simulink model "commhdlQPSKTxRx"  (R2025b)
settings: Solver=FixedStepDiscrete  StartTime=0.0  StopTime=stopTime  RelTol=1e-3
PostLoadFcn:
  | hScopeConfig = get_param([gcs '/Receiver/QPSK Rx/Frequency and Time Synchronizer/Symbol Synchronizer/No HDL/QPSK Receiver Eye Diagram'],'ScopeConfiguration');
  | 
  | hScopeConfig.OpenAtSimulationStart = false;
  | hScopeConfig.Visible = false;
  | SamplesPerSymbol = 4;
  | %UpsamplesRx = 1;
  | clear hScopeConfig
InitFcn:
  | commhdlQPSKTxRxModelInit;
  | % Rate bridge: ADRV9002/Jupiter radio runs at 15.36 MHz = 2x the 7.68 MHz
  | % (4 samples/symbol @ Rsym=1.92 MHz) the QPSK Rx requires. The deployed
  | % Receiver must downsample the ADC stream by 2. UpsamplesRx=1 fed the QPSK
  | % Rx 8 sps (2x-upsampled) and broke symbol sync / the loopback bit check.
  | UpsamplesRx = 1;   %% T8 RATE FIX: rail 15.36e6 == ADC bus rate,
  | %% no ingress decimation (was 2 when the rail sat on the 7.68e6 rung)
  | UpsamplesTx = 1;
  | clear simTimingOffset;
StopFcn:
  | if exist('simTimingOffset','var')
  |   disp('Simulation completed');
  |   %QPSKTxRxVerification;
  | end
undefined symbols (not defined in the file or in its folder): Add, Config, fsym, randsrc, RandStream, Rsym, Shift
libraries: hdlsllib x76, simulink x21, dspsigops x19, dsphdlfiltering2 x3, dsphdlsigops2 x2, dsphdlmathfun2 x2, commdigbbndpm3 x2, commchan3 x1, commrflib2 x1
(part 1 of 4)
CloseFcn:
  | clear Config CSLatency dataBits dataIn DBPP DescramblerLatency endLoc ...
  |         errSym errWaveform falsePacketsNo FCLatency idx initFramesNotToCompareInRx ...
  |         Nframes nReceivedBits PALatency PDLatency pktNo QPSKDemodLatency ...
  |         refQPSKSym refTxWaveform Rsym RxBits RxOut RxOutEnd RxOutSrt ...
  |         simAfterCS simBeforeSS simPeakFind simQPSKSym simSyncedPackets ...
  |         simTimingOffset simTxWaveform srtLoc SSLatency stopTime tout trueOffset ...
  |         TxBits validIn vPktNo
  | clear SamplesPerSymbol nErrBits nErrPkts nMissedPkts TxSymbolsMaxError TxWaveformMaxError
settings Model: DataTypeOverride=Off  Creator=The MathWorks, Inc.  LastModifiedBy=tcollins
settings SolverCC: AlgebraicLoopSolver=TrustRegion  MaxZcPerStep=1.0
settings DataIOCC: ReturnWorkspaceOutputs=off
settings OptimizationCC: BlockReduction=off  ConditionallyExecuteInputs=off  DefaultParameterBehavior=Inlined  ReuseModelBlockBuffer=off
settings DebuggingCC: AlgebraicLoopMsg=error  SingleTaskRateTransMsg=error  UnconnectedInputMsg=warning  UnconnectedOutputMsg=warning  UnconnectedLineMsg=warning  SubsystemReferenceDiagnosticForUnitTest=warning
settings HardwareCC: ProdBitPerPointer=32.0  ProdBitPerSizeT=32.0  ProdBitPerPtrDiffT=32.0  ProdLargestAtomicFloat=None  ProdIntDivRoundTo=Undefined  ProdEndianess=Unspecified  ProdWordSize=32.0  ProdHWDeviceType=ASIC/FPGA->ASIC/FPGA  TargetBitPerLong=64.0  TargetBitPerPointer=64.0  TargetBitPerSizeT=64.0  TargetBitPerPtrDiffT=64.0  TargetLongLongMode=on  TargetIntDivRoundTo=Zero  TargetEndianess=LittleEndian  TargetWordSize=64.0  TargetHWDeviceType=Custom Processor->MATLAB Host Computer  ProdEqTarget=off
settings ModelReferenceCC: EnableRefExpFcnMdlSchedulingChecks=on
settings RTWCC: GPUComputeCapability=3.5  DLArmComputeVersion=19.05

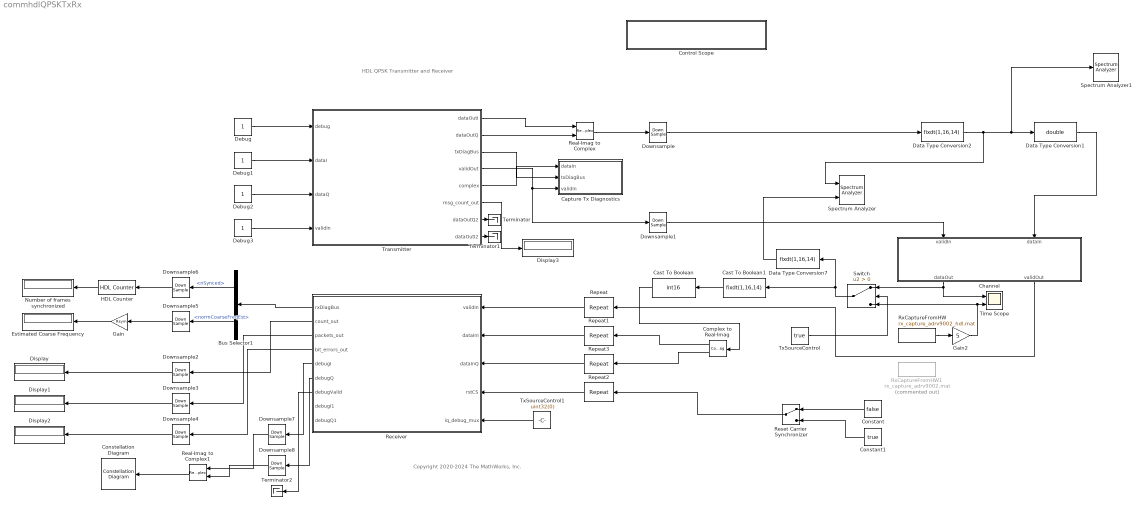
== system commhdlQPSKTxRx ==
  note: HDL QPSK Transmitter and Receiver
  note: Copyright 2020-2024 The MathWorks, Inc.
  Bus Selector1 : BusSelector  OutputSignals=nSynced,normCoarseFreqEst
  Capture Tx Diagnostics : Subsystem
  Cast To Boolean : DataTypeConversion  OutDataTypeStr=int16  ConvertRealWorld=Stored Integer (SI)  SaturateOnIntegerOverflow=off  RndMeth=Floor
  Cast To Boolean1 : DataTypeConversion  OutDataTypeStr=fixdt(1,16,14)  SaturateOnIntegerOverflow=off  RndMeth=Floor
  Channel : Subsystem  mask{EbN0dB=40, CFO=1e3, CPO=135, fractionalTimingOffset=0.55, timingFrequencyOffset=2}
      mask prompts: EbN0dB "Eb/N0 (in dB) :"; CFO "Carrier Frequency Offset (in Hz):"; CPO "Carrier Phase Offset (in Degrees) :"; fractionalTimingOffset "Fractional Timing Offset ( <1 ) :"; timingFrequencyOffset "Timing Frequency Offset (in PPM) :"
      mask init:
      | validateattributes(fractionalTimingOffset,{'double'},{'finite','scalar','nonnegative','>=',0,'<',1},'','fractionalTimingOffset');
      | validateattributes(timingFrequencyOffset,{'double'},{'finite','scalar','nonnegative'},'','timingFrequencyOffset');
      | validateattributes(EbN0dB,{'double'},{'scalar'},'','EbN0dB');
      | validateattributes(CFO,{'double'},{'finite','scalar',},'','CFO');
      | validateattributes(CPO,{'double'},{'finite','scalar'},'','CPO');
      | 
      | BitsPerSymbol = 2;      % QPSK
      | EbN0          = 10^(EbN0dB/10);
      | EsN0          = BitsPerSymbol*EbN0;
      | noiseVariance = 1/EsN0;  % QPSK symbol energy is normalized to 1 i.e. Es = 1
      | 
      | clear BitsPersymbol EbN0 EsN0
      settings: PortSchema="{\"entries\":[{\"content\":{\"sides\":[{\"content\":{\"connectorIds\":[]},\"type\":\"ConnectorPlacement.EquallySpacedRectSide\",\"uuid\":\"aa9ac445-3d73-401b-8e6c-a43fa6f53e3e\"},{\"content\":{\"connectorIds\":[],\"side\":\"RIGHT\"},\"type\":\"ConnectorPlacement.EquallySpacedRectSide\",\"uuid\":\"c8fbe2c1-ad18-4b81-8824-4fece19db9b5\"},{\"content\":{\"connectorIds\":[\"In1\",\"In2\"],\"side\":\"TOP\"},\"type\":\"ConnectorPlacement.EquallySpacedRectSide\",\"uuid\":\"2fdd8701-02b7-4a19-ab6e-54d2593732fa\"},{\"content\":{\"connectorIds\":[\"Out1\",\"Out2\"],\"side\":\"BOTTOM\"},\"type\":\"ConnectorPlacement.EquallySpacedRectSide\",\"uuid\":\"bd6ca111-71ba-47de-a918-1bcd41b09175\"}]},\"type\":\"ConnectorPlacement.EquallySpacedConnector\",\"uuid\":\"c410269f-5de3-4a8f-bc07-850237ff35fb\"}],\"packageUris\":[\"http://schema.mathworks.com/mf0/Connector/R2020b\"],\"version\":\"1.0\"}"
      mask DialogControl DescGroupVar Prompt: Channel
      mask Display: disp(['Double-Click' newline 'to set channel']);
  Complex to Real-Imag : ComplexToRealImag
  Constant : Constant  Value=false  SampleTime=1/(Rsym*Config.SamplesPerSymbol)
  Constant1 : Constant  Value=true  SampleTime=1/(Rsym*Config.SamplesPerSymbol)
  Constellation Diagram : ConstellationDiagram  WindowPosition=[594.000000,164.000000,600.000000,600.000000,]  Visible=on  ScopeFrameLocation=window  SymbolsToDisplaySource=Property  SymbolsToDisplay=1000  XLimits=[-1.375,8542.5]  YLimits=[-1.375,8542.5]  AxesLimits=[-1.375,8542.5]  MaximizeAxes=on  DefaultConfigurationName=comm.scopes.ConstellationDiagramBlockCfg
  Control Scope : Subsystem
      settings: OpenFcn=|
      | hScopeConfig1 = get_param([gcs '/Capture Tx Diagnostics/QPSK Transmitter Constellations'],'ScopeConfiguration');
      | hScopeConfig2 = get_param([gcs '/QPSK Rx/Frequency and Time Synchronizer/Symbol Synchronizer/No HDL/QPSK Receiver Eye Diagram'],'ScopeConfiguration');
      | hScopeConfig3 = get_param([gcs '/QPSK Rx/Frequency and Time Synchronizer/Symbol Synchronizer/No HDL/No HDL/QPSK Receiver Constellation 1'],'ScopeConfiguration');
      | hScopeConfig4 = get_param([gcs '/QPSK Rx/Frequency and Time Synchronizer/No HDL/QPSK Receiver Constellations 2'],'ScopeConfiguration');
      | hScopeConfig5 = get_param([gcs '/QPSK Rx/Frequency and Time Synchronizer/Preamble Detector/No HDL/Correlation Time Scope'],'ScopeConfiguration');
      | 
      | 
      | 
      | if all([hScopeConfig1.Visible hScopeConfig2.Visible hScopeConfig3.Visible hScopeConfig4.Visible hScopeConfig5.Visible])
      |    hScopeConfig1.Visible = false;
      |    hScopeConfig2.Visible = false;
      |    hScopeConfig3.Visible = false;
      |    hScopeConfig4.Visible = false;
      |    hScopeConfig5.Visible = false;
      | else
      |    hScopeConfig1.Visible = true;
      |    hScopeConfig2.Visible = true;
      |    hScopeConfig3.Visible = true;
      |    hScopeConfig4.Visible = true;
      |    hScopeConfig5.Visible = true;
      | end
      | 
      | clear hScopeConfig1 hScopeConfig2 hScopeConfig3 hScopeConfig4 hScopeConfig5;
      mask Display: disp('Double-click to turn on/off the Scopes');
  Data Type Conversion1 : DataTypeConversion  OutDataTypeStr=double  SaturateOnIntegerOverflow=off  RndMeth=Floor
  Data Type Conversion2 : DataTypeConversion  OutDataTypeStr=fixdt(1,16,14)  ConvertRealWorld=Stored Integer (SI)  SaturateOnIntegerOverflow=off  RndMeth=Floor
  Data Type Conversion7 : DataTypeConversion  OutDataTypeStr=fixdt(1,16,14)  SaturateOnIntegerOverflow=off  RndMeth=Floor
  Debug : Constant  OutDataTypeStr=uint32  SampleTime=-1
  Debug1 : Constant  OutDataTypeStr=int16  SampleTime=-1
  Debug2 : Constant  OutDataTypeStr=int16  SampleTime=-1
  Debug3 : Constant  OutDataTypeStr=boolean  SampleTime=-1
  Display{,1..3} (4 alike) : Display
  Downsample : DownSample  N=UpsamplesTx  RateOptions=Allow multirate processing
  Downsample1 : DownSample  N=UpsamplesTx  RateOptions=Allow multirate processing
  Downsample{2..8} (7 alike) : DownSample  N=UpsamplesRx  RateOptions=Allow multirate processing
  Estimated Coarse Frequency : Display
  Gain : Gain  Gain=Rsym
  Gain2 : Gain  Gain=5
  HDL Counter : hdlsllib/Sources/HDL Counter  CountType=Free running  CountInit=0  CountStep=1  CountMax=25  CountFromType=Initial value  CountFrom=0  CountResetPort=off  CountLoadPort=off  CountEnbPort=on  CountDirPort=off  CountHitOutputPort=off  CountDataType=Unsigned  CountWordLen=32  CountFracLen=0  CountSampTime=1
  Number of frames synchronized : Display
  Real-Imag to Complex : RealImagToComplex
  Real-Imag to Complex1 : RealImagToComplex
  Receiver : Subsystem  TreatAsAtomicUnit=on
  Repeat{,1..3} (4 alike) : dspsigops/Repeat  FactorSource=Dialog parameter  N=UpsamplesRx  Nmax=16  InputProcessing=Columns as channels (frame based)  RateOptions=Allow multirate processing  ic=0  mode=Unused parameter value
      settings: LibrarySourceBlock=commsequence2/Repeat
  Reset Carrier Synchronizer : ManualSwitch
  RxCaptureFromHW : FromFile  FileName=rx_capture_adrv9002_hdl.mat  OutDataTypeStr=double  SampleTime=1/(Rsym*Config.SamplesPerSymbol)  ExtrapolationBeforeFirstDataPoint=Hold first value  InterpolationWithinTimeRange=Zero order hold  ExtrapolationAfterLastDataPoint=Hold last value
  RxCaptureFromHW1 : FromFile  Commented=on  FileName=rx_capture_adrv9002.mat  OutDataTypeStr=double  SampleTime=1/(Rsym*Config.SamplesPerSymbol)  ExtrapolationBeforeFirstDataPoint=Hold first value  InterpolationWithinTimeRange=Zero order hold  ExtrapolationAfterLastDataPoint=Hold last value
  Spectrum Analyzer : SpectrumAnalyzer  NumInputPorts=2  WindowPosition=[494.000000,214.000000,800.000000,500.000000,]  Visible=on  ScopeFrameLocation=window  WindowInvariantSamplesPerUpdate=on  Span=7680000  StartFrequency=-3840000  StopFrequency=3840000  YLimits=[-47.9968 8.4452]
  Spectrum Analyzer1 : SpectrumAnalyzer  WindowPosition=[494.000000,214.000000,800.000000,500.000000,]  Visible=on  ScopeFrameLocation=window  WindowInvariantSamplesPerUpdate=on  Span=7680000  StartFrequency=-3840000  StopFrequency=3840000  YLimits=[-71.5508 10.9276]
  Switch : Switch  Criteria=u2 > Threshold  SaturateOnIntegerOverflow=off  InputSameDT=off
  Terminator : Terminator
  Terminator1 : Terminator
  Terminator2 : Terminator
  Time Scope : Scope  NumInputPorts=2
      settings: TimeUnits=Metric (based on Time Span)  ActiveDisplayYMinimum=-1.0052287666621835  ActiveDisplayYMaximum=0.87958747263253323  YLabel=Amplitude
  Transmitter : Subsystem  TreatAsAtomicUnit=on
  TxSourceControl : Constant  Value=true  SampleTime=-1
  TxSourceControl1 : Constant  Value=uint32(0)  SampleTime=-1
  wires:
  Bus Selector1/1 -> Downsample6/1  "<nSynced>"
  HDL Counter/1 -> Number of frames synchronized/1
  Bus Selector1/2 -> Downsample5/1  "<normCoarseFreqEst>"
  Gain/1 -> Estimated Coarse Frequency/1
  Data Type Conversion1/1 -> Channel/2(dataIn)
  Constant/1 -> Reset Carrier Synchronizer/1
  Constant1/1 -> Reset Carrier Synchronizer/2
  Channel/1(dataOut) -> Time Scope/1, Switch/1
  Switch/1 -> Data Type Conversion7/1, Cast To Boolean1/1
  TxSourceControl/1 -> Switch/2
  RxCaptureFromHW/1 -> Gain2/1
  Gain2/1 -> Switch/3, Time Scope/2
  Transmitter/4(validOut) -> Downsample1/1, Capture Tx Diagnostics/3(validIn)
  Transmitter/3(txDiagBus) -> Capture Tx Diagnostics/2(txDiagBus)
  Debug/1 -> Transmitter/1(debug)
  Channel/2(validOut) -> Repeat/1
  Reset Carrier Synchronizer/1 -> Repeat2/1
  Receiver/2(count_out) -> Downsample2/1
  Receiver/3(packets_out) -> Downsample3/1
  Receiver/4(bit_errors_out) -> Downsample4/1
  Debug2/1 -> Transmitter/3(dataQ)
  Debug1/1 -> Transmitter/2(dataI)
  Debug3/1 -> Transmitter/4(validIn)
  Transmitter/1(dataOutI) -> Real-Imag to Complex/1
  Transmitter/2(dataOutQ) -> Real-Imag to Complex/2
  Real-Imag to Complex/1 -> Downsample/1
  Transmitter/5(complex) -> Capture Tx Diagnostics/1(dataIn)
  Data Type Conversion2/1 -> Spectrum Analyzer/1, Spectrum Analyzer1/1, Data Type Conversion1/1
  Transmitter/6(msg_count_out) -> Display3/1
  Downsample/1 -> Data Type Conversion2/1
  Downsample1/1 -> Channel/1(validIn)
  Repeat/1 -> Receiver/1(validIn)
  Repeat1/1 -> Receiver/2(dataInI)
  Repeat2/1 -> Receiver/4(rstCS)
  Downsample2/1 -> Display/1
  Downsample3/1 -> Display1/1
  Downsample4/1 -> Display2/1
  Receiver/1(rxDiagBus) -> Bus Selector1/1
  Downsample5/1 -> Gain/1
  Downsample6/1 -> HDL Counter/1
  Transmitter/7(dataOutQ2) -> Terminator/1
  Transmitter/8(dataOutI2) -> Terminator1/1
  TxSourceControl1/1 -> Receiver/5(iq_debug_mux)
  Complex to Real-Imag/1 -> Repeat1/1
  Complex to Real-Imag/2 -> Repeat3/1
  Data Type Conversion7/1 -> Spectrum Analyzer/2
  Cast To Boolean/1 -> Complex to Real-Imag/1
  Repeat3/1 -> Receiver/3(dataInQ)
  Cast To Boolean1/1 -> Cast To Boolean/1
  Receiver/5(debugI) -> Downsample7/1
  Receiver/6(debugQ) -> Downsample8/1
  Downsample7/1 -> Real-Imag to Complex1/1
  Downsample8/1 -> Real-Imag to Complex1/2
  Real-Imag to Complex1/1 -> Constellation Diagram/1
  Receiver/7(debugValid) -> Terminator2/1

== system commhdlQPSKTxRx/Capture Tx Diagnostics ==
  dataIn : Inport
  txDiagBus : Inport  Port=2
  validIn : Inport  Port=3
  Bus Selector : BusSelector  OutputSignals=QPSKConstellationPoints,QPSKConstellationValid
  Data Type Conversion : DataTypeConversion  OutDataTypeStr=double  SaturateOnIntegerOverflow=off  RndMeth=Floor
  Data Type Conversion1 : DataTypeConversion  OutDataTypeStr=double  SaturateOnIntegerOverflow=off  RndMeth=Floor
  QPSK Transmitter Constellations : ConstellationDiagram  NumInputPorts=2  WindowPosition=[708.000000,285.000000,372.000000,357.000000,]  Visible=on  ScopeFrameLocation=window  SymbolsToDisplaySource=Property  SymbolsToDisplay=10000  ReferenceConstellation="{[0.70711+0.70711i        -0.70711+0.70711i        -0.70711-0.70711i         0.70711-0.70711i],[0.70711+0.70711i        -0.70711+0.70711i        -0.70711-0.70711i         0.70711-0.70711i]}"  ReferenceMarker={''o'',''o''}  ReferenceColor={[1 0 0],[1 0 0]}  XLimits=[-0.94638 0.94638]  YLimits=[-0.94638 0.94638]  AxesLimits=[-0.94638 0.94638]  ShowLegend=on  DefaultConfigurationName=comm.scopes.ConstellationDiagramBlockCfg
      settings: OpenAtSimulationStart=off
  Subsystem : Subsystem
  Subsystem1 : Subsystem
  Unit Delay Enabled Synchronous : hdlsllib/Discrete/Unit Delay Enabled Synchronous  InitialCondition=0.0  SampleTime=-1
  Unit Delay Enabled Synchronous1 : hdlsllib/Discrete/Unit Delay Enabled Synchronous  InitialCondition=0.0  SampleTime=-1
  wires:
  txDiagBus/1 -> Bus Selector/1
  Bus Selector/1 -> Data Type Conversion/1  "<QPSKConstellationPoints>"
  Data Type Conversion/1 -> Unit Delay Enabled Synchronous/1, Subsystem/1(In1)
  dataIn/1 -> Data Type Conversion1/1
  Bus Selector/2 -> Subsystem/Enable, Unit Delay Enabled Synchronous/2  "<QPSKConstellationValid>"
  Data Type Conversion1/1 -> Unit Delay Enabled Synchronous1/1, Subsystem1/1(In1)
  validIn/1 -> Subsystem1/Enable, Unit Delay Enabled Synchronous1/2
  Unit Delay Enabled Synchronous1/1 -> QPSK Transmitter Constellations/2  "RRC Filtered Output"
  Unit Delay Enabled Synchronous/1 -> QPSK Transmitter Constellations/1  "Modulator Output"

== system commhdlQPSKTxRx/Channel ==
  validIn : Inport
  dataIn : Inport  Port=2
  AWGN Channel : commchan3/AWGN Channel  LegacyMode=on  NoiseMethod="Signal to noise ratio  (SNR)"  noiseMode=Variance from mask  EbNo=EbN0dB  EsNo=10  SNR=10  BitsPerSymbol=2  SignalPower=1  SpecifySymbolPeriod=off  SamplesPerSymbol=1  SymbolPeriod=1/fsym  VarianceSource=Parameter  Variance=noiseVariance  RandomStream=Global stream  Seed=67  SimulateUsing=Code generation
  Add : Sum  Inputs=|++
  Add1 : Sum  Inputs=++|
  Constant : Constant  Value=fractionalTimingOffset  SampleTime=-1
  Constant1 : Constant  Value=timingFrequencyOffset * 1e-6  SampleTime=-1
  Delay : Delay  DelayLength=1
  Mod 1 : Subsystem
  Phase/ Frequency Offset : commrflib2/Phase// Frequency Offset  phaseOffset=CPO  freqPort=off  freqOffset=CFO
  Variable Fractional Delay : dspsigops/Variable Fractional Delay  mode=OBSOLETE  modeActive=Linear  L=4  FarrowL=4  R=10  alpha=1  dmax=100  InputProcessing=Columns as channels (frame based)  ic=0  noDFT=off  fallbackFIR=Clip to the minimum value necessary for centered kernel  fallbackFarrow=Clip to the minimum value necessary for centered kernel  roundingMode=Zero  overflowMode=off
  dataOut : Outport
  validOut : Outport  Port=2
  wires:
  AWGN Channel/1 -> Phase/ Frequency Offset/1
  Variable Fractional Delay/1 -> AWGN Channel/1
  dataIn/1 -> Variable Fractional Delay/1
  Constant1/1 -> Add/1
  Delay/1 -> Add/2, Add1/2
  Add/1 -> Delay/1
  Add1/1 -> Mod 1/1(In1)
  Constant/1 -> Add1/1
  Mod 1/1(Out1) -> Variable Fractional Delay/2
  Phase/ Frequency Offset/1 -> dataOut/1
  validIn/1 -> validOut/1

== system commhdlQPSKTxRx/Control Scope ==

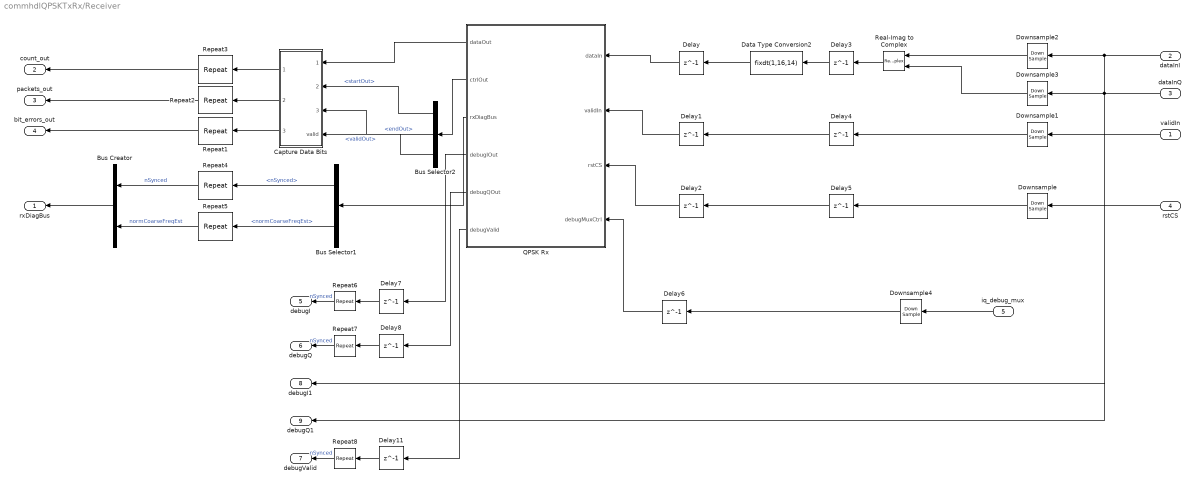
== system commhdlQPSKTxRx/Receiver ==
  validIn : Inport
  dataInI : Inport  Port=2
  dataInQ : Inport  Port=3
  rstCS : Inport  Port=4
  iq_debug_mux : Inport  Port=5  OutDataTypeStr=uint32
  Bus Creator : BusCreator  Inputs=2
  Bus Selector1 : BusSelector  OutputSignals=nSynced,normCoarseFreqEst
  Bus Selector2 : BusSelector  OutputSignals=startOut,endOut,validOut
  Capture Data Bits : Subsystem
  Data Type Conversion2 : DataTypeConversion  OutDataTypeStr=fixdt(1,16,14)  ConvertRealWorld=Stored Integer (SI)  SaturateOnIntegerOverflow=off  RndMeth=Floor
  Delay{,1..8,11} (10 alike) : Delay  DelayLength=1
  Downsample{,1..4} (5 alike) : DownSample  N=UpsamplesRx  RateOptions=Allow multirate processing
  QPSK Rx : Subsystem
      mask init:
      | integAvgLen = 2^15;
      | 
      | RxParams            = commhdlQPSKTxRxParameters();
      | Preamble            = RxParams.Preamble;
      | QPSKConstellation   = RxParams.QPSKConstellation;
      | dataBitsPerPacket   = RxParams.DataBitsPerPacket;
      | SamplesPerSymbol    = RxParams.SamplesPerSymbol;
      | RRCCoef             = RxParams.RRCCoef;
      | bitsPerPacket        = RxParams.BitsPerPacket;
      | 
      | rxPreambleMFCoeffs  = RxParams.rxPreambleMFCoeffs;
      | preambleSymbols     = RxParams.preambleSymbols;
      | ThresoldGainFac     = RxParams.ThresoldGainFac;
      | 
      | % AGC Parameters
      | AGCReference           = RxParams.AGCReference;
      | AGCLoopGain            = RxParams.AGCLoopGain;
      | 
      | % CS parameters
      | CSKp                   = RxParams.CSKp;
      | CSK0                   = RxParams.CSK0;  
      | CSLoopFilterPropGain   = RxParams.CSLoopFilterPropGain;
      | CSLoopFilterIntegGain  = RxParams.CSLoopFilterIntegGain;
      | CFOChangeDetectThreshold = RxParams.CFOChangeDetectThreshold;
      | 
      | % SS parameters
      | SSKp                   = RxParams.SSKp; 
      | SSK0                   = RxParams.SSK0;  
      | SSLoopFilterPropGain   = RxParams.SSLoopFilterPropGain;
      | SSLoopFilterIntegGain  = RxParams.SSLoopFilterIntegGain;
      | 
      | % preamble detector parameters
      | searchSamples          = RxParams.SearchSamples;
      | 
      | clear RxParams;
  Real-Imag to Complex : RealImagToComplex
  Repeat{1..8} (8 alike) : dspsigops/Repeat  FactorSource=Dialog parameter  N=UpsamplesRx  Nmax=16  InputProcessing=Columns as channels (frame based)  RateOptions=Allow multirate processing  ic=0  mode=Unused parameter value
      settings: LibrarySourceBlock=commsequence2/Repeat
  rxDiagBus : Outport
  count_out : Outport  Port=2
  packets_out : Outport  Port=3
  bit_errors_out : Outport  Port=4
  debugI : Outport  Port=5
  debugQ : Outport  Port=6
  debugValid : Outport  Port=7
  debugI1 : Outport  Port=8
  debugQ1 : Outport  Port=9
  wires:
  Bus Selector2/1 -> Capture Data Bits/2(dataSrt)  "<startOut>"
  QPSK Rx/1(dataOut) -> Capture Data Bits/1(dataOut)
  QPSK Rx/2(ctrlOut) -> Bus Selector2/1
  Bus Selector2/2 -> Capture Data Bits/3(dataEnd)  "<endOut>"
  rstCS/1 -> Downsample/1
  validIn/1 -> Downsample1/1
  Bus Selector2/3 -> Capture Data Bits/4(valid)  "<validOut>"
  Capture Data Bits/1(count_out) -> Repeat3/1
  Capture Data Bits/2(packets_out) -> Repeat2/1
  Capture Data Bits/3(bit_errors_out) -> Repeat1/1
  Downsample1/1 -> Delay4/1
  Repeat1/1 -> bit_errors_out/1
  Repeat2/1 -> packets_out/1
  Repeat3/1 -> count_out/1
  QPSK Rx/3(rxDiagBus) -> Bus Selector1/1
  Bus Creator/1 -> rxDiagBus/1
  Bus Selector1/1 -> Repeat4/1  "<nSynced>"
  Bus Selector1/2 -> Repeat5/1  "<normCoarseFreqEst>"
  Repeat4/1 -> Bus Creator/1  "nSynced"
  Repeat5/1 -> Bus Creator/2  "normCoarseFreqEst"
  dataInQ/1 -> debugQ1/1, Downsample3/1
  dataInI/1 -> debugI1/1, Downsample2/1
  Real-Imag to Complex/1 -> Delay3/1
  Downsample2/1 -> Real-Imag to Complex/1
  Downsample3/1 -> Real-Imag to Complex/2
  Data Type Conversion2/1 -> Delay/1
  Delay/1 -> QPSK Rx/1(dataIn)
  Delay1/1 -> QPSK Rx/2(validIn)
  Delay2/1 -> QPSK Rx/3(rstCS)
  Delay3/1 -> Data Type Conversion2/1
  Delay4/1 -> Delay1/1
  Delay5/1 -> Delay2/1
  QPSK Rx/4(debugIOut) -> Delay7/1
  QPSK Rx/5(debugQOut) -> Delay8/1
  Repeat6/1 -> debugI/1  "nSynced"
  Repeat7/1 -> debugQ/1  "nSynced"
  iq_debug_mux/1 -> Downsample4/1
  Delay6/1 -> QPSK Rx/4(debugMuxCtrl)
  Downsample4/1 -> Delay6/1
  Repeat8/1 -> debugValid/1  "nSynced"
  QPSK Rx/6(debugValid) -> Delay11/1
  Delay7/1 -> Repeat6/1
  Delay8/1 -> Repeat7/1
  Delay11/1 -> Repeat8/1
  Downsample/1 -> Delay5/1

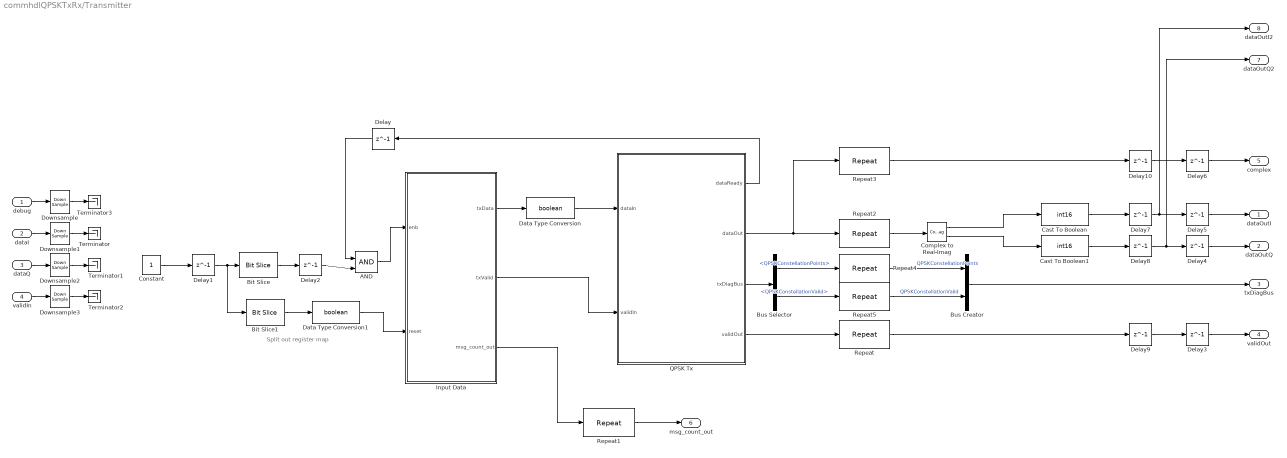
== system commhdlQPSKTxRx/Transmitter ==
  note: Split out register map
  debug : Inport  PortDimensions=1
  dataI : Inport  Port=2
  dataQ : Inport  Port=3
  validIn : Inport  Port=4
  AND : Logic  IconShape=distinctive  AllPortsSameDT=off  OutDataTypeStr=boolean
  Bit Slice : hdlsllib/Logic and Bit Operations/Bit Slice  lidx=0  ridx=0
  Bit Slice1 : hdlsllib/Logic and Bit Operations/Bit Slice  lidx=1  ridx=1
  Bus Creator : BusCreator  Inputs=2
  Bus Selector : BusSelector  OutputSignals=QPSKConstellationPoints,QPSKConstellationValid
  Cast To Boolean : DataTypeConversion  OutDataTypeStr=int16  ConvertRealWorld=Stored Integer (SI)  SaturateOnIntegerOverflow=off  RndMeth=Floor
  Cast To Boolean1 : DataTypeConversion  OutDataTypeStr=int16  ConvertRealWorld=Stored Integer (SI)  SaturateOnIntegerOverflow=off  RndMeth=Floor
  Complex to Real-Imag : ComplexToRealImag
  Constant : Constant  OutDataTypeStr=uint32  SampleTime=-1
  Data Type Conversion : DataTypeConversion  OutDataTypeStr=boolean  SaturateOnIntegerOverflow=off  RndMeth=Floor
  Data Type Conversion1 : DataTypeConversion  OutDataTypeStr=boolean  SaturateOnIntegerOverflow=off  RndMeth=Floor
  Delay{,1..10} (11 alike) : Delay  DelayLength=1
  Downsample{,1..3} (4 alike) : DownSample  N=UpsamplesTx  RateOptions=Allow multirate processing
  Input Data : Subsystem  mask{dataBits=reshape(repmat(randsrc(2240*1,1,[0,1],RandStream('mcg16807','Seed',0)), 59,1), [2240*59,1]), Rsym=3.84e6}
      mask prompts: dataBits "Data Bits :"; Rsym "Symbol Rate (in baud rate)  :"
      mask Display: disp(['Double-Click' newline 'to set data bits']);
  QPSK Tx : Subsystem
      mask init:
      | TxParams           = commhdlQPSKTxRxParameters();
      | Preamble            = TxParams.Preamble;
      | QPSKConstellation   = TxParams.QPSKConstellation;
      | dataBitsPerPacket   = TxParams.DataBitsPerPacket;
      | SamplesPerSymbol    = TxParams.SamplesPerSymbol;
      | RRCCoef             = TxParams.RRCCoef;
      | dataRAMAddrWidth    = TxParams.txDataRAMAddrWidth;
      | bitsPerPacket       = TxParams.BitsPerPacket;
      | 
      | clear TxParams;
  Repeat{,1..5} (6 alike) : dspsigops/Repeat  FactorSource=Dialog parameter  N=UpsamplesTx  Nmax=16  InputProcessing=Columns as channels (frame based)  RateOptions=Allow multirate processing  ic=0  mode=Unused parameter value
      settings: LibrarySourceBlock=commsequence2/Repeat
  Terminator{,1..3} (4 alike) : Terminator
  dataOutI : Outport
  dataOutQ : Outport  Port=2
  txDiagBus : Outport  Port=3
  validOut : Outport  Port=4
  complex : Outport  Port=5
  msg_count_out : Outport  Port=6
  dataOutQ2 : Outport  Port=7
  dataOutI2 : Outport  Port=8
  wires:
  Input Data/2(txValid) -> QPSK Tx/2(validIn)
  Input Data/1(txData) -> Data Type Conversion/1
  Data Type Conversion/1 -> QPSK Tx/1(dataIn)
  QPSK Tx/4(validOut) -> Repeat/1
  QPSK Tx/1(dataReady) -> Delay/1
  AND/1 -> Input Data/1(enb)
  Bit Slice/1 -> Delay2/1
  Delay/1 -> AND/1
  Delay1/1 -> Bit Slice1/1, Bit Slice/1
  Delay2/1 -> AND/2
  Bit Slice1/1 -> Data Type Conversion1/1
  Data Type Conversion1/1 -> Input Data/2(reset)
  dataI/1 -> Downsample1/1
  dataQ/1 -> Downsample2/1
  validIn/1 -> Downsample3/1
  Constant/1 -> Delay1/1
  debug/1 -> Downsample/1
  QPSK Tx/2(dataOut) -> Repeat3/1, Repeat2/1
  Complex to Real-Imag/1 -> Cast To Boolean/1
  Complex to Real-Imag/2 -> Cast To Boolean1/1
  Input Data/3(msg_count_out) -> Repeat1/1
  Repeat/1 -> Delay9/1
  Repeat2/1 -> Complex to Real-Imag/1
  Repeat3/1 -> Delay10/1
  Downsample/1 -> Terminator3/1
  Downsample1/1 -> Terminator/1
  Downsample2/1 -> Terminator1/1
  Downsample3/1 -> Terminator2/1
  Repeat1/1 -> msg_count_out/1
  QPSK Tx/3(txDiagBus) -> Bus Selector/1
  Bus Selector/1 -> Repeat4/1  "<QPSKConstellationPoints>"
  Repeat4/1 -> Bus Creator/1  "QPSKConstellationPoints"
  Bus Selector/2 -> Repeat5/1  "<QPSKConstellationValid>"
  Repeat5/1 -> Bus Creator/2  "QPSKConstellationValid"
  Bus Creator/1 -> txDiagBus/1
  Cast To Boolean/1 -> Delay7/1
  Cast To Boolean1/1 -> Delay8/1
  Delay3/1 -> validOut/1
  Delay4/1 -> dataOutQ/1
  Delay5/1 -> dataOutI/1
  Delay6/1 -> complex/1
  Delay7/1 -> dataOutI2/1, Delay5/1
  Delay8/1 -> dataOutQ2/1, Delay4/1
  Delay9/1 -> Delay3/1
  Delay10/1 -> Delay6/1

== system commhdlQPSKTxRx/Capture Tx Diagnostics/Subsystem ==
  In1 : Inport
  Enable : EnablePort
  To Workspace : ToWorkspace  VariableName=simQPSKSym  SampleTime=-1
      settings: Save2DSignal=2-D array (concatenate along first dimension)
  wires:
  In1/1 -> To Workspace/1

== system commhdlQPSKTxRx/Capture Tx Diagnostics/Subsystem1 ==
  In1 : Inport
  Enable : EnablePort
  To Workspace1 : ToWorkspace  VariableName=simTxWaveform  SampleTime=-1
      settings: Save2DSignal=2-D array (concatenate along first dimension)
  wires:
  In1/1 -> To Workspace1/1

== system commhdlQPSKTxRx/Channel/Mod 1 ==
  In1 : Inport
  Constant : Constant  SampleTime=-1
  Mod : Math  Operator=mod
  Out1 : Outport
  wires:
  Mod/1 -> Out1/1
  In1/1 -> Mod/1
  Constant/1 -> Mod/2

== system commhdlQPSKTxRx/Receiver/Capture Data Bits ==
  dataOut : Inport
  dataSrt : Inport  Port=2
  dataEnd : Inport  Port=3
  valid : Inport  Port=4
  Display : Display
  Display1 : Display
  Display2 : Display
  MATLAB Function : MATLAB Function  TreatAsAtomicUnit=on
  To Workspace : ToWorkspace  VariableName=RxOut  SampleTime=-1
      settings: Save2DSignal=2-D array (concatenate along first dimension)
  To Workspace1 : ToWorkspace  VariableName=RxOutSrt  SampleTime=-1
      settings: Save2DSignal=2-D array (concatenate along first dimension)
  To Workspace2 : ToWorkspace  VariableName=RxOutEnd  SampleTime=-1
      settings: Save2DSignal=2-D array (concatenate along first dimension)
  count_out : Outport
  packets_out : Outport  Port=2
  bit_errors_out : Outport  Port=3
  wires:
  dataOut/1 -> MATLAB Function/2(datain), To Workspace/1
  dataSrt/1 -> MATLAB Function/3(start), To Workspace1/1
  dataEnd/1 -> MATLAB Function/4(stop), To Workspace2/1
  valid/1 -> MATLAB Function/1(valid)
  MATLAB Function/1(count_out) -> count_out/1, Display/1
  MATLAB Function/2(packets_out) -> packets_out/1, Display1/1
  MATLAB Function/3(bit_errors_out) -> bit_errors_out/1, Display2/1

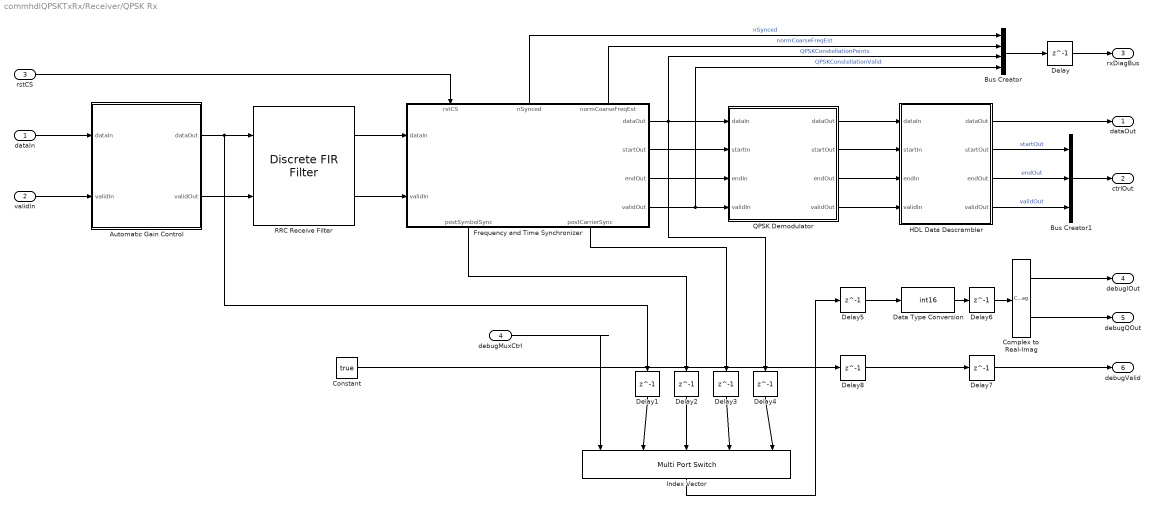
== system commhdlQPSKTxRx/Receiver/QPSK Rx ==
  dataIn : Inport  OutDataTypeStr=fixdt(1,16,14)  PortDimensions=1  SampleTime=1/(Rsym*SamplesPerSymbol)
      settings: SignalType=complex
  validIn : Inport  Port=2  OutDataTypeStr=boolean  PortDimensions=1  SampleTime=1/(Rsym*SamplesPerSymbol)
  rstCS : Inport  Port=3  OutDataTypeStr=boolean  PortDimensions=1
      settings: SignalType=complex
  debugMuxCtrl : Inport  Port=4  OutDataTypeStr=uint32  PortDimensions=1  SampleTime=1/(Rsym*SamplesPerSymbol)
  Automatic Gain Control : Subsystem  mask{Ref=AGCReference, LFG=AGCLoopGain}
      mask prompts: Ref "Error Detector Reference:"; LFG "Loop Filter Gain"
  Bus Creator : BusCreator  Inputs=4
  Bus Creator1 : BusCreator  Inputs=3
  Complex to Real-Imag : ComplexToRealImag
  Constant : Constant  Value=true  SampleTime=1/(Rsym*SamplesPerSymbol)
  Data Type Conversion : DataTypeConversion  OutDataTypeStr=int16  ConvertRealWorld=Stored Integer (SI)  SaturateOnIntegerOverflow=off  RndMeth=Floor
  Delay{,1..8} (9 alike) : Delay  DelayLength=1
  Frequency and Time Synchronizer : Subsystem
      settings: PortSchema="{\"entries\":[{\"content\":{\"sides\":[{\"content\":{\"connectorIds\":[\"In1\",\"In2\"]},\"type\":\"ConnectorPlacement.EquallySpacedRectSide\",\"uuid\":\"8bc6a452-5111-4806-8ca9-335cb622aea6\"},{\"content\":{\"connectorIds\":[\"Out1\",\"Out2\",\"Out3\",\"Out4\"],\"side\":\"RIGHT\"},\"type\":\"ConnectorPlacement.EquallySpacedRectSide\",\"uuid\":\"b0f43c98-f5c0-4f62-94ae-d69789942eef\"},{\"content\":{\"connectorIds\":[\"In3\",\"Out7\",\"Out8\"],\"side\":\"TOP\"},\"type\":\"ConnectorPlacement.EquallySpacedRectSide\",\"uuid\":\"427ff3b3-b896-4008-9584-d311480df763\"},{\"content\":{\"connectorIds\":[\"Out5\",\"Out6\"],\"side\":\"BOTTOM\"},\"type\":\"ConnectorPlacement.EquallySpacedRectSide\",\"uuid\":\"f704cb90-80a1-4198-8b72-e70182b45e73\"},{\"content\":{\"side\":\"HIDDEN\"},\"type\":\"ConnectorPlacement.EquallySpacedRectSide\",\"uuid\":\"f6309498-1e43-486f-b6b5-2c6570711f8e\"}]},\"type\":\"ConnectorPlacement.EquallySpacedConnector\",\"uuid\":\"f0ce492e-c9e1-4b35-98ef-84d77b696cfe\"}],\"packageUris\":[\"http://schema.mathworks.com/mf0/Connector/R2020b\"],\"version\":\"1.0\"}"
  HDL Data Descrambler : Subsystem
  Index Vector : MultiPortSwitch  DataPortOrder=Zero-based contiguous  Inputs=4  DiagnosticForDefault=None  zeroidx=on  SaturateOnIntegerOverflow=off  InputSameDT=off
  QPSK Demodulator : Subsystem
  RRC Receive Filter : dsphdlfiltering2/Discrete FIR Filter  NumeratorSource=Property  Numerator=RRCCoef  NumeratorPrototype=[]  FilterStructure=Direct form systolic  SerializationOption=Minimum number of cycles between valid input samples  NumCycles=2  NumberOfMultipliers=2  SimulateUsing=Code generation  roundingMode=Floor  overflowMode=off  CoefficientsDataTypeStr=Inherit: Same word length as input  OutputDataTypeStr=Inherit: Same word length as input  ResetInputPort=off  HDLGlobalReset=off  CoeffMultiplier=Multiplier  UseMultForPow2Coeff=on  FrameInputSymmOptim=off
  dataOut : Outport
  ctrlOut : Outport  Port=2
  rxDiagBus : Outport  Port=3
  debugIOut : Outport  Port=4
  debugQOut : Outport  Port=5
  debugValid : Outport  Port=6
  wires:
  rstCS/1 -> Frequency and Time Synchronizer/3(rstCS)
  QPSK Demodulator/1(dataOut) -> HDL Data Descrambler/1(dataIn)
  validIn/1 -> Automatic Gain Control/2(validIn)
  Automatic Gain Control/2(validOut) -> RRC Receive Filter/2
  RRC Receive Filter/1 -> Frequency and Time Synchronizer/1(dataIn)
  HDL Data Descrambler/3(endOut) -> Bus Creator1/2  "endOut"
  QPSK Demodulator/3(endOut) -> HDL Data Descrambler/3(endIn)
  Frequency and Time Synchronizer/8(normCoarseFreqEst) -> Bus Creator/2  "normCoarseFreqEst"
  Bus Creator1/1 -> ctrlOut/1
  HDL Data Descrambler/2(startOut) -> Bus Creator1/1  "startOut"
  Frequency and Time Synchronizer/3(endOut) -> QPSK Demodulator/3(endIn)
  RRC Receive Filter/2 -> Frequency and Time Synchronizer/2(validIn)
  Frequency and Time Synchronizer/7(nSynced) -> Bus Creator/1  "nSynced"
  Bus Creator/1 -> Delay/1
  Automatic Gain Control/1(dataOut) -> Delay1/1, RRC Receive Filter/1
  Frequency and Time Synchronizer/1(dataOut) -> Delay4/1, QPSK Demodulator/1(dataIn), Bus Creator/3  "QPSKConstellationPoints"
  dataIn/1 -> Automatic Gain Control/1(dataIn)
  HDL Data Descrambler/1(dataOut) -> dataOut/1
  HDL Data Descrambler/4(validOut) -> Bus Creator1/3  "validOut"
  QPSK Demodulator/2(startOut) -> HDL Data Descrambler/2(startIn)
  Frequency and Time Synchronizer/2(startOut) -> QPSK Demodulator/2(startIn)
  Frequency and Time Synchronizer/4(validOut) -> QPSK Demodulator/4(validIn), Bus Creator/4  "QPSKConstellationValid"
  QPSK Demodulator/4(validOut) -> HDL Data Descrambler/4(validIn)
  Delay/1 -> rxDiagBus/1
  Frequency and Time Synchronizer/5(postSymbolSync) -> Delay2/1
  Frequency and Time Synchronizer/6(postCarrierSync) -> Delay3/1
  debugMuxCtrl/1 -> Index Vector/1
  Complex to Real-Imag/2 -> debugQOut/1
  Complex to Real-Imag/1 -> debugIOut/1
  Data Type Conversion/1 -> Delay6/1
  Delay1/1 -> Index Vector/2
  Delay2/1 -> Index Vector/3
  Delay3/1 -> Index Vector/4
  Delay4/1 -> Index Vector/5
  Delay5/1 -> Data Type Conversion/1
  Index Vector/1 -> Delay5/1
  Delay6/1 -> Complex to Real-Imag/1
  Delay7/1 -> debugValid/1
  Delay8/1 -> Delay7/1
  Constant/1 -> Delay8/1

== system commhdlQPSKTxRx/Transmitter/Input Data ==
  enb : Inport
  reset : Inport  Port=2
  Cast To Boolean : DataTypeConversion  OutDataTypeStr=boolean  SaturateOnIntegerOverflow=off  RndMeth=Floor
  Delay : Delay  DelayLength=1
  Display : Display
  Message Generator : Subsystem
  Terminator : Terminator
  Terminator1 : Terminator
  txData : Outport
  txValid : Outport  Port=2
  msg_count_out : Outport  Port=3
  wires:
  Message Generator/4(valid) -> txValid/1
  Message Generator/1(out) -> txData/1
  enb/1 -> Message Generator/2(enable)
  Message Generator/5(count) -> Display/1
  Message Generator/2(stop) -> Delay/1
  Delay/1 -> Cast To Boolean/1
  Cast To Boolean/1 -> Message Generator/1(reset)
  reset/1 -> Terminator/1
  Message Generator/3(start) -> Terminator1/1
  Message Generator/6(msg_count_out) -> msg_count_out/1

== system commhdlQPSKTxRx/Transmitter/QPSK Tx ==
  dataIn : Inport  OutDataTypeStr=boolean  PortDimensions=1
  validIn : Inport  Port=2  OutDataTypeStr=boolean  PortDimensions=1
  Bit Packetizer : Subsystem
  Bus Creator : BusCreator  Inputs=2
  HDL Data Scrambler : Subsystem
  QPSK Modulator : Subsystem
  RRC Transmit Filter : Subsystem
  dataReady : Outport
  dataOut : Outport  Port=2
  txDiagBus : Outport  Port=3
  validOut : Outport  Port=4
  wires:
  validIn/1 -> Bit Packetizer/2(validIn)
  RRC Transmit Filter/2(validOut) -> validOut/1
  HDL Data Scrambler/1(dataOut) -> QPSK Modulator/1(dataIn)
  Bit Packetizer/1(bitsOut) -> HDL Data Scrambler/1(dataIn)
  QPSK Modulator/2(validOut) -> Bus Creator/2, RRC Transmit Filter/2(validIn)  "QPSKConstellationValid"
  dataIn/1 -> Bit Packetizer/1(dataIn)
  Bit Packetizer/3(dataEnd) -> HDL Data Scrambler/3(endIn)
  HDL Data Scrambler/2(validOut) -> QPSK Modulator/2(validIn)
  RRC Transmit Filter/1(dataOut) -> dataOut/1
  QPSK Modulator/1(dataOut) -> Bus Creator/1, RRC Transmit Filter/1(dataIn)  "QPSKConstellationPoints"
  Bit Packetizer/2(dataStart) -> HDL Data Scrambler/2(startIn)
  Bit Packetizer/5(dataReady) -> dataReady/1
  Bus Creator/1 -> txDiagBus/1
  Bit Packetizer/4(bitsValid) -> HDL Data Scrambler/4(validIn)

== system commhdlQPSKTxRx/Receiver/QPSK Rx/Automatic Gain Control ==
  dataIn : Inport
  validIn : Inport  Port=2
  Data Type Conversion : DataTypeConversion  OutDataTypeStr=fixdt(1,16,10)  SaturateOnIntegerOverflow=off  RndMeth=Floor
  Delay{1..5} (5 alike) : Delay
  Error Detector : Subsystem
  Loop Filter : Subsystem
  Product : Product  OutDataTypeStr=Inherit: Same as first input
  dataOut : Outport
  validOut : Outport  Port=2
  wires:
  Data Type Conversion/1 -> Delay1/1
  Delay5/1 -> Delay3/1
  Delay3/1 -> validOut/1
  Delay4/1 -> Product/1
  Delay1/1 -> Product/2
  Loop Filter/1(gain) -> Data Type Conversion/1
  Error Detector/1(err) -> Loop Filter/1(err)
  validIn/1 -> Delay5/1
  Delay2/1 -> Error Detector/1(dataIn), dataOut/1
  dataIn/1 -> Delay4/1
  Product/1 -> Delay2/1

== system commhdlQPSKTxRx/Receiver/QPSK Rx/Frequency and Time Synchronizer ==
  dataIn : Inport
  validIn : Inport  Port=2
  rstCS : Inport  Port=3
  Carrier Synchronizer : Subsystem
      settings: PortSchema="{\"entries\":[{\"content\":{\"sides\":[{\"content\":{\"connectorIds\":[\"In1\",\"In2\",\"In3\"]},\"type\":\"ConnectorPlacement.EquallySpacedRectSide\",\"uuid\":\"ee58e5dc-083a-48cb-b7f3-66ed8a15890f\"},{\"content\":{\"connectorIds\":[\"Out1\",\"Out2\"],\"side\":\"RIGHT\"},\"type\":\"ConnectorPlacement.EquallySpacedRectSide\",\"uuid\":\"6d121164-5065-4840-a82e-fa57a8e9650e\"},{\"content\":{\"connectorIds\":[\"In4\"],\"side\":\"TOP\"},\"type\":\"ConnectorPlacement.EquallySpacedRectSide\",\"uuid\":\"54d2b8e3-f516-4572-94a0-c914196ae8e4\"}]},\"type\":\"ConnectorPlacement.EquallySpacedConnector\",\"uuid\":\"0f2a6472-efd0-42ca-a030-ab436081b5e1\"}],\"packageUris\":[\"http://schema.mathworks.com/mf0/Connector/R2020b\"],\"version\":\"1.0\"}"
  Coarse Frequency Compensator : Subsystem
      settings: PortSchema="{\"entries\":[{\"content\":{\"sides\":[{\"content\":{\"connectorIds\":[\"In1\",\"In2\"]},\"type\":\"ConnectorPlacement.EquallySpacedRectSide\",\"uuid\":\"138aa5bd-62db-47d6-b55f-f529a6004434\"},{\"content\":{\"connectorIds\":[\"Out1\",\"Out2\",\"Out3\"],\"side\":\"RIGHT\"},\"type\":\"ConnectorPlacement.EquallySpacedRectSide\",\"uuid\":\"8e6ccec0-f736-48ab-be6d-feac886e083d\"},{\"content\":{\"connectorIds\":[\"Out4\"],\"side\":\"TOP\"},\"type\":\"ConnectorPlacement.EquallySpacedRectSide\",\"uuid\":\"d4535392-74fa-432a-a39c-b98ba26e8163\"},{\"content\":{\"side\":\"BOTTOM\"},\"type\":\"ConnectorPlacement.EquallySpacedRectSide\",\"uuid\":\"770ac6a2-7a02-4a77-858b-592982deaf6e\"}]},\"type\":\"ConnectorPlacement.EquallySpacedConnector\",\"uuid\":\"a9b944be-f88b-4ab6-a5e1-6824362eb9ca\"}],\"packageUris\":[\"http://schema.mathworks.com/mf0/Connector/R2020b\"],\"version\":\"1.0\"}"
  No HDL : Subsystem
      settings: PortSchema="{\"entries\":[{\"content\":{\"sides\":[{\"content\":{\"connectorIds\":[\"In1\",\"In2\"]},\"type\":\"ConnectorPlacement.EquallySpacedRectSide\",\"uuid\":\"df96a46d-149f-4580-adf6-e5cf26cffa9b\"},{\"content\":{\"connectorIds\":[\"In3\",\"In4\"],\"side\":\"RIGHT\"},\"type\":\"ConnectorPlacement.EquallySpacedRectSide\",\"uuid\":\"1c46d09c-cb37-4618-ac4e-e5ef50df41fb\"},{\"content\":{\"connectorIds\":[],\"side\":\"TOP\"},\"type\":\"ConnectorPlacement.EquallySpacedRectSide\",\"uuid\":\"7fe62300-46d7-4234-a31d-eecffed4f6e6\"},{\"content\":{\"connectorIds\":[],\"side\":\"BOTTOM\"},\"type\":\"ConnectorPlacement.EquallySpacedRectSide\",\"uuid\":\"05ecd563-28f5-4cfd-b718-5032a7458763\"}]},\"type\":\"ConnectorPlacement.EquallySpacedConnector\",\"uuid\":\"4b3d5859-a469-4389-9e5d-e5f07416a9a1\"}],\"packageUris\":[\"http://schema.mathworks.com/mf0/Connector/R2020b\"],\"version\":\"1.0\"}"
  Packet Controller : Subsystem
  Phase Ambiguity Estimation and Correction : Subsystem
  Preamble Detector : Subsystem
  Symbol Synchronizer : Subsystem
  dataOut : Outport
  startOut : Outport  Port=2
  endOut : Outport  Port=3
  validOut : Outport  Port=4
  postSymbolSync : Outport  Port=5
  postCarrierSync : Outport  Port=6
  nSynced : Outport  Port=7
  normCoarseFreqEst : Outport  Port=8
  wires:
  Coarse Frequency Compensator/3(validOut) -> Carrier Synchronizer/3(validIn)
  Coarse Frequency Compensator/1(dataOut) -> Carrier Synchronizer/1(dataIn)
  Phase Ambiguity Estimation and Correction/1(dataOut) -> Packet Controller/1(dataIn)
  Phase Ambiguity Estimation and Correction/3(validOut) -> Packet Controller/3(validIn)
  Symbol Synchronizer/2(validOut) -> No HDL/2(In2), Coarse Frequency Compensator/2(validIn)
  Symbol Synchronizer/1(dataOut) -> postSymbolSync/1, No HDL/1(In1), Coarse Frequency Compensator/1(dataIn)
  Phase Ambiguity Estimation and Correction/2(syncPulseOut) -> Packet Controller/2(syncPulse)
  Preamble Detector/3(validOut) -> Phase Ambiguity Estimation and Correction/3(validIn)
  Preamble Detector/1(dataOut) -> Phase Ambiguity Estimation and Correction/1(dataIn)
  validIn/1 -> Symbol Synchronizer/2(validIn)
  dataIn/1 -> Symbol Synchronizer/1(dataIn)
  Coarse Frequency Compensator/2(rstCS) -> Carrier Synchronizer/2(internalRst)
  Packet Controller/1(dataOut) -> dataOut/1
  Packet Controller/2(startOut) -> startOut/1
  Packet Controller/3(endOut) -> endOut/1
  Packet Controller/4(validOut) -> validOut/1
  Preamble Detector/2(syncPulse) -> nSynced/1, Phase Ambiguity Estimation and Correction/2(syncPulseIn)
  Carrier Synchronizer/1(dataOut) -> postCarrierSync/1, No HDL/3(In3), Preamble Detector/1(dataIn)
  Carrier Synchronizer/2(validOut) -> No HDL/4(In4), Preamble Detector/2(validIn)
  Coarse Frequency Compensator/4(normalizedFreqEst) -> normCoarseFreqEst/1
  rstCS/1 -> Carrier Synchronizer/4(manualRst)

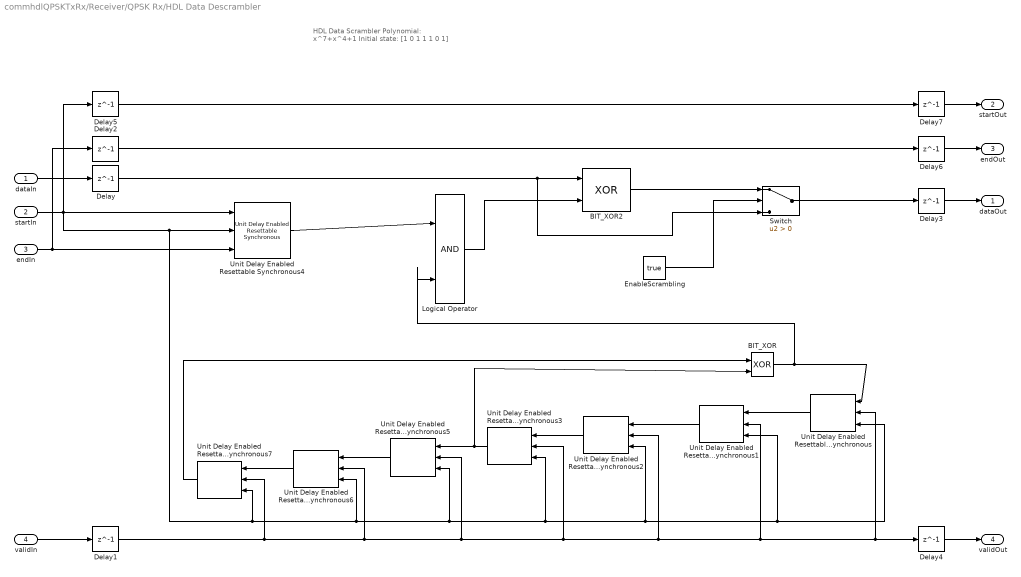
== system commhdlQPSKTxRx/Receiver/QPSK Rx/HDL Data Descrambler ==
  note: HDL Data Scrambler
      | Polynomial: x^7+x^4+1
      | Initial state: [1 0 1 1 1 0 1]
  dataIn : Inport
  startIn : Inport  Port=2
  endIn : Inport  Port=3
  validIn : Inport  Port=4
  BIT_XOR : Logic  Operator=XOR  IconShape=distinctive  AllPortsSameDT=off  OutDataTypeStr=boolean
  BIT_XOR2 : Logic  Operator=XOR  IconShape=distinctive  AllPortsSameDT=off  OutDataTypeStr=boolean
  Delay{,1..7} (8 alike) : Delay  DelayLength=1
  EnableScrambling : Constant  Value=true  SampleTime=-1
  Logical Operator : Logic  IconShape=distinctive  AllPortsSameDT=off  OutDataTypeStr=boolean
  Switch : Switch  Criteria=u2 > Threshold  SaturateOnIntegerOverflow=off  InputSameDT=off
  Unit Delay Enabled Resettable Synchronous{,2..3,5,7} (5 alike) : hdlsllib/Discrete/Unit Delay Enabled Resettable Synchronous  InitialCondition=1  SampleTime=-1
  Unit Delay Enabled Resettable Synchronous1 : hdlsllib/Discrete/Unit Delay Enabled Resettable Synchronous  InitialCondition=0  SampleTime=-1
  Unit Delay Enabled Resettable Synchronous4 : hdlsllib/Discrete/Unit Delay Enabled Resettable Synchronous  InitialCondition=0  SampleTime=-1
  Unit Delay Enabled Resettable Synchronous6 : hdlsllib/Discrete/Unit Delay Enabled Resettable Synchronous  InitialCondition=0.0  SampleTime=-1
  dataOut : Outport  InitialOutput=0
  startOut : Outport  Port=2  InitialOutput=0
  endOut : Outport  Port=3  InitialOutput=0
  validOut : Outport  Port=4  InitialOutput=0
  wires:
  Delay4/1 -> validOut/1
  Delay3/1 -> dataOut/1
  endIn/1 -> Delay2/1, Unit Delay Enabled Resettable Synchronous4/3
  Logical Operator/1 -> BIT_XOR2/2
  Unit Delay Enabled Resettable Synchronous4/1 -> Logical Operator/1
  Delay1/1 -> Unit Delay Enabled Resettable Synchronous6/2, Unit Delay Enabled Resettable Synchronous2/2, Unit Delay Enabled Resettable Synchronous1/2, Unit Delay Enabled Resettable Synchronous/2, Delay4/1, Unit Delay Enabled Resettable Synchronous3/2, Unit Delay Enabled Resettable Synchronous5/2, Unit Delay Enabled Resettable Synchronous7/2
  Delay/1 -> Switch/3, BIT_XOR2/1
  startIn/1 -> Delay5/1, Unit Delay Enabled Resettable Synchronous4/1, Unit Delay Enabled Resettable Synchronous4/2, Unit Delay Enabled Resettable Synchronous6/3, Unit Delay Enabled Resettable Synchronous5/3, Unit Delay Enabled Resettable Synchronous1/3, Unit Delay Enabled Resettable Synchronous/3, Unit Delay Enabled Resettable Synchronous2/3, Unit Delay Enabled Resettable Synchronous3/3, Unit Delay Enabled Resettable Synchronous7/3
  dataIn/1 -> Delay/1
  validIn/1 -> Delay1/1
  BIT_XOR/1 -> Unit Delay Enabled Resettable Synchronous/1, Logical Operator/2
  Unit Delay Enabled Resettable Synchronous1/1 -> Unit Delay Enabled Resettable Synchronous2/1
  Unit Delay Enabled Resettable Synchronous2/1 -> Unit Delay Enabled Resettable Synchronous3/1
  Unit Delay Enabled Resettable Synchronous/1 -> Unit Delay Enabled Resettable Synchronous1/1
  Unit Delay Enabled Resettable Synchronous3/1 -> BIT_XOR/2, Unit Delay Enabled Resettable Synchronous5/1
  Unit Delay Enabled Resettable Synchronous5/1 -> Unit Delay Enabled Resettable Synchronous6/1
  Unit Delay Enabled Resettable Synchronous6/1 -> Unit Delay Enabled Resettable Synchronous7/1
  Unit Delay Enabled Resettable Synchronous7/1 -> BIT_XOR/1
  Delay2/1 -> Delay6/1
  Delay5/1 -> Delay7/1
  Delay6/1 -> endOut/1
  Delay7/1 -> startOut/1
  EnableScrambling/1 -> Switch/2
  BIT_XOR2/1 -> Switch/1
  Switch/1 -> Delay3/1

== system commhdlQPSKTxRx/Receiver/QPSK Rx/QPSK Demodulator ==
  dataIn : Inport
  startIn : Inport  Port=2
  endIn : Inport  Port=3
  validIn : Inport  Port=4
  Delay{,1..13} (14 alike) : Delay  DelayLength=1
  QPSK Demodulator Baseband : commdigbbndpm3/QPSK Demodulator Baseband  OutType=Bit  DecType=Hard decision  VarSource=Dialog  Variance=1  Dec=Gray  Ph=pi/4  outDtype1=boolean  outDtype2=Inherit via internal rule  derotateFactorWordLen=16  derotateFactorDataTypeStr=Inherit: Same word length as input  derotateFactorLastDataTypeStr=Inherit: Same word length as input
  Serializer : Subsystem
  Signal Specification : SignalSpecification  Dimensions=1
  dataOut : Outport
  startOut : Outport  Port=2
  endOut : Outport  Port=3
  validOut : Outport  Port=4
  wires:
  Delay/1 -> QPSK Demodulator Baseband/1
  Delay1/1 -> Delay5/1
  Delay6/1 -> Delay4/1
  Delay7/1 -> Delay13/1
  Delay2/1 -> Delay6/1
  Delay3/1 -> Delay7/1
  Signal Specification/1 -> Delay/1
  QPSK Demodulator Baseband/1 -> Delay12/1
  Delay8/1 -> dataOut/1
  Delay9/1 -> validOut/1
  Delay10/1 -> startOut/1
  Delay11/1 -> endOut/1
  Delay5/1 -> Serializer/2(In2)
  Delay12/1 -> Serializer/1(u)
  Delay4/1 -> Delay10/1
  Delay13/1 -> Delay11/1
  Serializer/1(Out1) -> Delay8/1
  Serializer/2(Out2) -> Delay9/1
  dataIn/1 -> Signal Specification/1
  validIn/1 -> Delay1/1
  startIn/1 -> Delay2/1
  endIn/1 -> Delay3/1

== system commhdlQPSKTxRx/Transmitter/Input Data/Message Generator ==
  reset : Inport
  enable : Inport  Port=2
  MATLAB Function : MATLAB Function  TreatAsAtomicUnit=on
  out : Outport
  stop : Outport  Port=2
  start : Outport  Port=3
  valid : Outport  Port=4
  count : Outport  Port=5
  msg_count_out : Outport  Port=6
  wires:
  MATLAB Function/3(stop) -> stop/1
  MATLAB Function/1(out) -> out/1
  reset/1 -> MATLAB Function/2(reset)
  MATLAB Function/2(start) -> start/1
  enable/1 -> MATLAB Function/1(enable)
  MATLAB Function/4(valid) -> valid/1
  MATLAB Function/5(count_out) -> count/1
  MATLAB Function/6(msg_count_out) -> msg_count_out/1

== system commhdlQPSKTxRx/Transmitter/QPSK Tx/Bit Packetizer ==
  dataIn : Inport
  validIn : Inport  Port=2
  Compare To Constant : hdlsllib/Logic and Bit Operations/Compare To Constant  relop===  const=length(Preamble)  OutDataTypeStr=boolean
  Compare To Constant1 : hdlsllib/Logic and Bit Operations/Compare To Constant  relop===  const=bitsPerPacket - 1  OutDataTypeStr=boolean
  Compare To Constant2 : hdlsllib/Logic and Bit Operations/Compare To Constant  relop=>=  const=length(Preamble)  OutDataTypeStr=boolean
  Data Bits FIFO : Subsystem
  Data Type Conversion : DataTypeConversion  OutDataTypeStr=boolean  SaturateOnIntegerOverflow=off  RndMeth=Floor
  DataReadyPaceCmp : simulink/Logic and Bit Operations/Compare To Constant  relop===  const=SamplesPerSymbol/2 - 1  OutDataTypeStr=boolean
  HDL Counter : hdlsllib/Sources/HDL Counter  CountType=Count limited  CountInit=0  CountStep=1  CountMax=SamplesPerSymbol/2 - 1  CountFromType=Initial value  CountFrom=0  CountResetPort=off  CountLoadPort=off  CountEnbPort=on  CountDirPort=off  CountHitOutputPort=off  CountDataType=Unsigned  CountWordLen=nextpow2(SamplesPerSymbol/2)  CountFracLen=0  CountSampTime=1
  Logical Operator : Logic  AllPortsSameDT=off  OutDataTypeStr=boolean
  Logical Operator1 : Logic  AllPortsSameDT=off  OutDataTypeStr=boolean
  Logical Operator2 : Logic  Operator=NOT  AllPortsSameDT=off  OutDataTypeStr=boolean
  Preamble Bits Generator : Subsystem
  Switch : Switch  Criteria=u2 ~= 0  SaturateOnIntegerOverflow=off  InputSameDT=off
  bitsOut : Outport
  dataStart : Outport  Port=2
  dataEnd : Outport  Port=3
  bitsValid : Outport  Port=4
  dataReady : Outport  Port=5
  wires:
  dataIn/1 -> Data Bits FIFO/1(data)
  validIn/1 -> Data Bits FIFO/2(push)
  Compare To Constant/1 -> Logical Operator/1
  Compare To Constant1/1 -> Logical Operator1/2
  Logical Operator/1 -> dataStart/1
  Logical Operator1/1 -> dataEnd/1
  Data Bits FIFO/5(fullRAM) -> Logical Operator2/1
  Logical Operator2/1 -> HDL Counter/1
  Data Bits FIFO/1(dataOut) -> Switch/1
  Data Bits FIFO/3(sampleCount) -> Preamble Bits Generator/2(sampleCount), Compare To Constant/1, Compare To Constant1/1, Compare To Constant2/1
  Data Bits FIFO/4(sampleCountValid) -> bitsValid/1, Logical Operator/2, Logical Operator1/1, Preamble Bits Generator/3(sampleCountValid)
  Data Bits FIFO/2(activeFrame) -> Preamble Bits Generator/1(activeFrame)
  Preamble Bits Generator/1(preambleBits) -> Switch/3
  Compare To Constant2/1 -> Switch/2
  Switch/1 -> bitsOut/1
  Data Type Conversion/1 -> dataReady/1
  HDL Counter/1 -> DataReadyPaceCmp/1
  DataReadyPaceCmp/1 -> Data Type Conversion/1
